simulink model "FOC_physical"  (R2024b)
settings: Solver=FixedStepAuto  StartTime=0.0  StopTime=3  FixedStep=1e-6  RelTol=1e-3
undefined symbols (not defined in the file): Down, GPTRIP1SEL, Ki_d, Ki_q, Ki_s, Kp_d, Kp_q, Kp_s, lambda, Ld, ma, p, T_max, TZ1, Up, Vdc
libraries: spsIGBTDiodeLib x6, simulink x4, spsCurrentMeasurementLib x3, spsDCVoltageSourceLib x1, spsPermanentMagnetSynchronousMachineLib x1, c2802xlib x1, eeStairGenerator x1, sps_lib x1
settings Model: Creator=ahmed  LastModifiedBy=ahmed
settings SolverCC: ZeroCrossAlgorithm=Adaptive
settings DebuggingCC: IgnoredZcDiagnostic=none

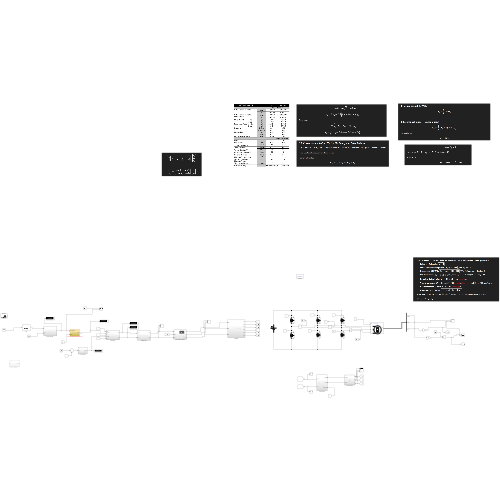
[thumbnail: Simulink's stored preview of the top-level diagram]
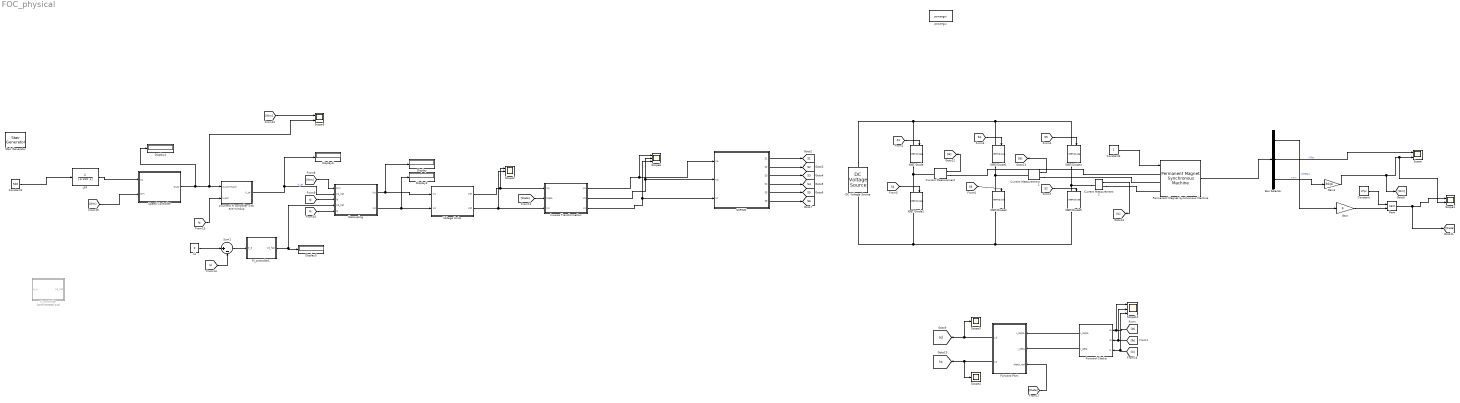
== system FOC_physical ==
  Bus Selector : BusSelector  OutputSignals=theta,Te,w
  Constant : Constant  Value=2*pi
  Constant1 : Constant  Value=500
  Constant3 : Constant
  Current Measurement : spsCurrentMeasurementLib/Current Measurement  PhasorSimulation=off  OutputType=Complex  PSBequivalent=0
  Current Measurement1 : spsCurrentMeasurementLib/Current Measurement  PhasorSimulation=off  OutputType=Complex  PSBequivalent=0
  Current Measurement2 : spsCurrentMeasurementLib/Current Measurement  PhasorSimulation=off  OutputType=Complex  PSBequivalent=0
  DC Voltage Source : spsDCVoltageSourceLib/DC Voltage Source  Amplitude=320  Measurements=None
  "Decoupling " : Subsystem
  Display{,3..6} (5 alike) : Display
  Forward Clacke : Subsystem
  Forward Park : Subsystem
  Gain : Gain  Gain=p
  Gain1 : Gain  Gain=30/pi
  IGBT/Diode{,1..5} (6 alike) : spsIGBTDiodeLib/IGBT//Diode  Ron=1e-3  Rs=1e5  Cs=inf  Measurements=on
  Id : Constant  Value=0
  Inverse Transformation : Subsystem
  LPF : TransferFcn  Denominator=[1/100 1]
  PI_controller : Subsystem  Commented=on
  PI_controller1 : Subsystem
  Permanent Magnet Synchronous Machine : spsPermanentMagnetSynchronousMachineLib/Permanent Magnet Synchronous Machine  NbPhases=3  FluxDistribution=Sinusoidal  RotorType=Round  MechanicalLoad=Torque Tm  PresetModel=No  ShowDetailedParameters=on  MeasurementBus=on  Resistance=1.45  Inductance=8.5e-3  dqInductances=[6.2e-3,6.2e-3]  La=6.2e-3  MachineConstant=Flux linkage established by magnets (V.s)  Flux=.0620  VoltageCst=44.9822  TorqueCst=0.372  Flat=120  Mechanical=[2.6e-5 9.55e-5 4 .03]  PolePairs=4  InitialConditions=[0,0, 0,0]  InitialConditions5ph=[0 0 0 0 0 0]  RefAngle=Aligned with phase A axis (original Park)  IterativeDiscreteModel=Trapezoidal non iterative  TsBlock=-1  TsPowergui=0
  Rem : Math  Operator=rem
  SVPWM : Subsystem
  Scope : Scope  NumInputPorts=2
  Scope1 : Scope  NumInputPorts=2
  Scope12 : Scope  NumInputPorts=3
  Scope2 : Scope  NumInputPorts=3
  Scope3 : Scope
  Scope4 : Scope
  Scope5 : Scope  NumInputPorts=2
  Scope6 : Scope  NumInputPorts=3
  "Speed Controller " : Subsystem
  Stair Generator : eeStairGenerator/Stair Generator  LabelModeActiveChoice=Discrete  TimeInput=[0 1 1.3 1.7 2 2.4]  AmplitudeInput=[200 1000 3000 4500 2000 0]  SampleTime=1e-6  RepeatPattern=off  OutDataTypeStr=double
      settings: LibrarySourceBlock=ee_sl_lib/General Control/Stair Generator
  Sum1 : Sum  Inputs=|+-
  Voltage limits : Subsystem
  powergui : sps_lib/powergui  Priority=1  SimulationMode=Continuous  SampleTime=1e-6  frequency=60  Iterations=50  frequencyindice=0  Pbase=100e6  ErrMax=1e-4  UnitsV=kV  UnitsW=MW  buscounter=0  FunctionMessages=off  echomessages=off  EnableUseOfTLC=off  CurrentSourceSwitches=off  DisableSnubberDevices=off  DisableRonSwitches=off  DisableVfSwitches=off  DisplayEquations=off  AutomaticDiscreteSolvers=off  SolverType=Tustin/Backward Euler (TBE)  Interpol=off  ExternalGateDelay=off  methode=off  Ts=100  x0status=blocks  SPID=on  SwTol=0  HookPort=off  NonlinearTolerance=1e-4  nMaxIteration=100  ContinueOnMaxIteration=off  RestoreLinks=warning  ResistiveCurrentMeasurement=off  Frange=[0:2:500]  Ylog=off  Xlog=on  ShowGrid=off  save=off  variable=ZData  structure=0  ZoomFFT=off  StartTime=0.0  cycles=1  DisplayStyle=1  fundamental=60  FreqAxis=off  MaxFrequency=1000  frequencyindicesteady=1  RmsSteady=1  display=off
  q-current PI controller with anti-windup : Subsystem
  tag scope: Id=global, Iq=global, S1=global, S2=global, S3=global, S4=global, S5=global, S6=global
  wires:
  Rem/1 -> Scope1/1, [theta]
  Permanent Magnet Synchronous Machine/1 -> Bus Selector/1
  Gain/1 -> Rem/2
  Constant/1 -> Rem/1
  [S3] -> IGBT/Diode1/1
  [S6] -> IGBT/Diode3/1
  [S5] -> IGBT/Diode4/1
  SVPWM/1(S1) -> [S1]
  SVPWM/2(S2) -> [S2]
  SVPWM/6(S6) -> [S6]
  SVPWM/4(S4) -> [S4]
  SVPWM/3(S3) -> [S3]
  SVPWM/5(S5) -> [S5]
  [S4] -> IGBT/Diode2/1
  [S1] -> IGBT/Diode/1
  [S2] -> IGBT/Diode5/1
  [Iq] -> "Decoupling "/5(Iq)
  "Decoupling "/2(Vd) -> Display3/1, Voltage limits/2(Vd)
  [Wm] -> Scope5/1
  Voltage limits/2(Vd*) -> Inverse Transformation/3(Vd), Scope2/2
  [Id] -> "Decoupling "/3(Id)
  PI_controller1/1(Vd_hat) -> "Decoupling "/4(Vd_hat), Display5/1
  Id/1 -> Sum1/1
  Inverse Transformation/1(Va) -> SVPWM/1(Va), Scope6/1
  Sum1/1 -> PI_controller1/1(e_d)
  "Decoupling "/1(Vq) -> Display/1, Voltage limits/1(Vq)
  Voltage limits/1(Vq*) -> Scope2/1, Inverse Transformation/1(Vq)
  "Speed Controller "/1(Out1) -> Display4/1, q-current PI controller with anti-windup/1(Iq command), Scope5/2
  Inverse Transformation/3(Vc) -> SVPWM/3(Vc), Scope6/3
  [theta] -> Inverse Transformation/2(theta)
  [Wm] -> "Decoupling "/1(Wm)
  Inverse Transformation/2(Vb) -> SVPWM/2(Vb), Scope6/2
  Constant3/1 -> Permanent Magnet Synchronous Machine/1
  [Id] -> Sum1/2
  [Wm] -> "Speed Controller "/2(Wm)
  Gain1/1 -> Scope1/2, Scope/2, [Wm]
  LPF/1 -> "Speed Controller "/1(In1)
  Forward Clacke/1(I_alpha) -> Forward Park/1(I_alpha)
  [theta] -> Forward Park/3(theta_rad)
  [Ib] -> Forward Clacke/2(Ib), Scope12/2
  Forward Park/1(I_d) -> [Id], Scope3/1
  [Ia] -> Forward Clacke/1(Ia), Scope12/1
  [Ic] -> Forward Clacke/3(Ic), Scope12/3
  Forward Park/2(I_q) -> [Iq], Scope4/1
  Forward Clacke/2(I_beta) -> Forward Park/2(I_beta)
  Current Measurement/1 -> [Ia]
  Current Measurement1/1 -> [Ib]
  Current Measurement2/1 -> [Ic]
  [Iq] -> q-current PI controller with anti-windup/2(Iq act)
  q-current PI controller with anti-windup/1(V_q*) -> Display6/1, "Decoupling "/2(Vq_hat)  "V_q*"
  Constant1/1 -> LPF/1
  Bus Selector/1 -> Gain/1  "<theta>"
  Bus Selector/2 -> Scope/1  "<Te>"
  Bus Selector/3 -> Gain1/1  "<w>"
  connections:
  DC Voltage Source/RConn1 -- IGBT/Diode4/LConn1 -- IGBT/Diode1/LConn1 -- IGBT/Diode/LConn1
  Current Measurement/LConn1 -- IGBT/Diode/RConn1 -- IGBT/Diode2/LConn1
  Current Measurement2/LConn1 -- IGBT/Diode4/RConn1 -- IGBT/Diode5/LConn1
  DC Voltage Source/LConn1 -- IGBT/Diode5/RConn1 -- IGBT/Diode3/RConn1 -- IGBT/Diode2/RConn1
  Current Measurement1/LConn1 -- IGBT/Diode1/RConn1 -- IGBT/Diode3/LConn1
  Current Measurement2/RConn1 -- Permanent Magnet Synchronous Machine/LConn3
  Current Measurement1/RConn1 -- Permanent Magnet Synchronous Machine/LConn2
  Current Measurement/RConn1 -- Permanent Magnet Synchronous Machine/LConn1

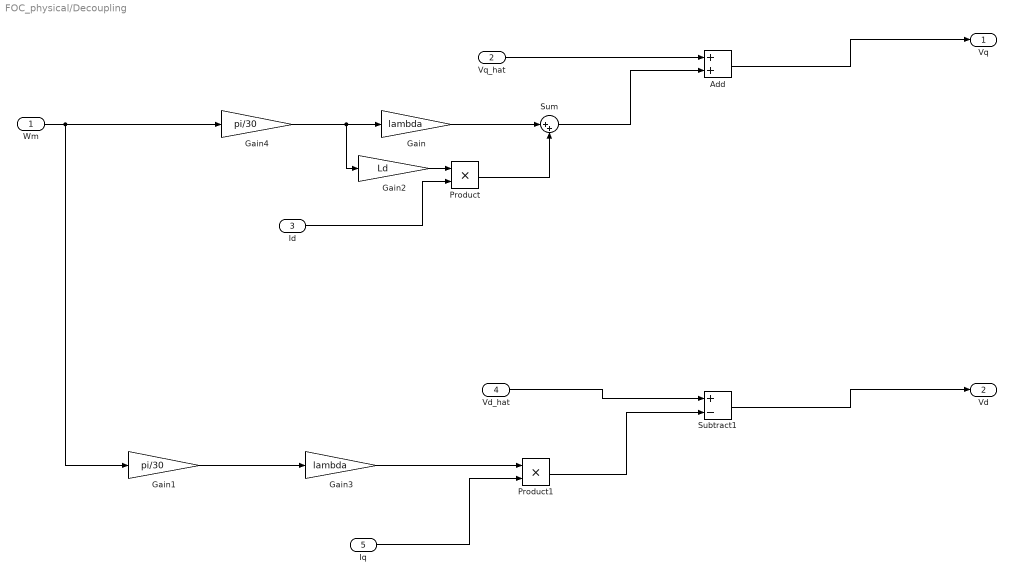
== system FOC_physical/Decoupling  ==
  Wm : Inport
  Vq_hat : Inport  Port=2
  Id : Inport  Port=3
  Vd_hat : Inport  Port=4
  Iq : Inport  Port=5
  Add : Sum
  Gain : Gain  Gain=lambda
  Gain1 : Gain  Gain=pi/30
  Gain2 : Gain  Gain=Ld
  Gain3 : Gain  Gain=lambda
  Gain4 : Gain  Gain=pi/30
  Product : Product
  Product1 : Product
  Subtract1 : Sum  Inputs=+-
  Sum : Sum  Inputs=|++
  Vq : Outport
  Vd : Outport  Port=2
  wires:
  Vq_hat/1 -> Add/1
  Vd_hat/1 -> Subtract1/1
  Gain2/1 -> Product/1
  Id/1 -> Product/2
  Product/1 -> Sum/2
  Gain/1 -> Sum/1
  Sum/1 -> Add/2
  Gain3/1 -> Product1/1
  Product1/1 -> Subtract1/2
  Iq/1 -> Product1/2
  Gain4/1 -> Gain2/1, Gain/1
  Add/1 -> Vq/1
  Subtract1/1 -> Vd/1
  Wm/1 -> Gain1/1, Gain4/1
  Gain1/1 -> Gain3/1

== system FOC_physical/Forward Clacke ==
  Ia : Inport
  Ib : Inport  Port=2
  Ic : Inport  Port=3
  Gain : Gain  Gain=0.5
  Gain1 : Gain  Gain=0.5
  Gain2 : Gain  Gain=2/3
  Gain3 : Gain  Gain=sqrt(3)/2
  Gain4 : Gain  Gain=2/3
  Sum : Sum  Inputs=+--
  Sum1 : Sum  Inputs=+-
  I_alpha : Outport
  I_beta : Outport  Port=2
  wires:
  Ib/1 -> Gain/1, Sum1/1
  Gain/1 -> Sum/2
  Gain2/1 -> I_alpha/1
  Sum1/1 -> Gain3/1
  Gain1/1 -> Sum/3
  Ic/1 -> Gain1/1, Sum1/2
  Sum/1 -> Gain2/1
  Gain3/1 -> Gain4/1
  Ia/1 -> Sum/1
  Gain4/1 -> I_beta/1

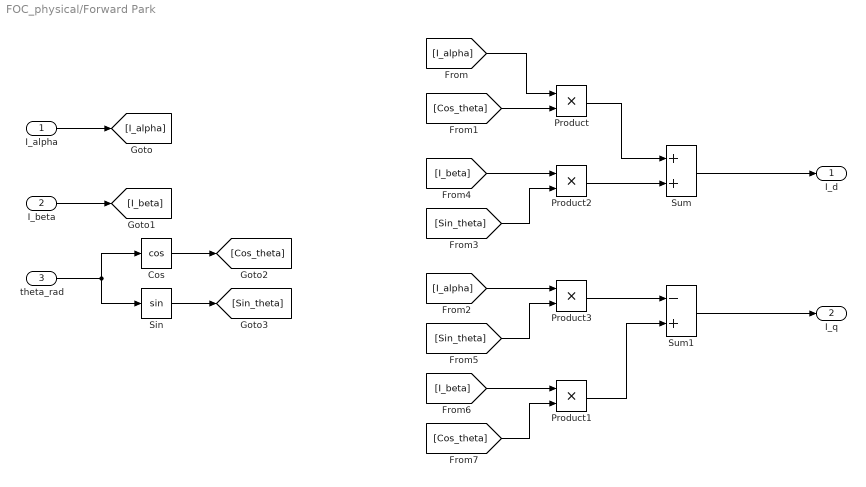
== system FOC_physical/Forward Park ==
  I_alpha : Inport
  I_beta : Inport  Port=2
  theta_rad : Inport  Port=3
  Cos : Trigonometry  Operator=cos
  Product{,1..3} (4 alike) : Product
  Sin : Trigonometry
  Sum : Sum
  Sum1 : Sum  Inputs=-+
  I_d : Outport
  I_q : Outport  Port=2
  wires:
  [Cos_theta] -> Product1/2
  [I_beta] -> Product1/1
  [Sin_theta] -> Product3/2
  [I_alpha] -> Product3/1
  Product1/1 -> Sum1/2
  [I_beta] -> Product2/1
  [Sin_theta] -> Product2/2
  [Cos_theta] -> Product/2
  Sin/1 -> [Sin_theta]
  Cos/1 -> [Cos_theta]
  theta_rad/1 -> Cos/1, Sin/1
  [I_alpha] -> Product/1
  I_beta/1 -> [I_beta]
  I_alpha/1 -> [I_alpha]
  Product3/1 -> Sum1/1
  Product2/1 -> Sum/2
  Product/1 -> Sum/1
  Sum1/1 -> I_q/1
  Sum/1 -> I_d/1

== system FOC_physical/Inverse Transformation ==
  Vq : Inport
  theta : Inport  Port=2
  Vd : Inport  Port=3
  "Inverse Park " : Subsystem
  inverse Clark : Subsystem
  Va : Outport
  Vb : Outport  Port=2
  Vc : Outport  Port=3
  wires:
  Vq/1 -> "Inverse Park "/3(In3)
  theta/1 -> "Inverse Park "/1(In1)
  Vd/1 -> "Inverse Park "/2(In2)
  "Inverse Park "/1(Valpha) -> inverse Clark/1(In1)
  "Inverse Park "/2(Vbeta) -> inverse Clark/2(In2)
  inverse Clark/1(Va) -> Va/1
  inverse Clark/2(Vb) -> Vb/1
  inverse Clark/3(Vc) -> Vc/1

== system FOC_physical/PI_controller ==
  note: Kp = ((2*zeta*wn)-(Rs/ld))*Ld
  note: Kp = (Wn^2)*Ld
  e_q : Inport
  Display : Display
  Integrator : Integrator
  Ki : Gain  Gain=Ki_q
  Kp : Gain  Gain=Kp_q
  Product : Product
  Scope : Scope
  Sum : Sum  Inputs=|++
  Vq_hat : Outport
  wires:
  Kp/1 -> Sum/1
  Sum/1 -> Display/1, Vq_hat/1
  e_q/1 -> Ki/1, Kp/1
  [Stop_q_integrator] -> Scope/1, Product/2
  Product/1 -> Integrator/1
  Integrator/1 -> Sum/2
  Ki/1 -> Product/1

== system FOC_physical/PI_controller1 ==
  e_d : Inport
  Integrator : Integrator
  Ki : Gain  Gain=Ki_d
  Kp : Gain  Gain=Kp_d
  Product : Product
  Sum : Sum  Inputs=|++
  Time Scope : Scope
  Vd_hat : Outport
  wires:
  Kp/1 -> Sum/1
  e_d/1 -> Ki/1, Kp/1
  Sum/1 -> Vd_hat/1
  Product/1 -> Integrator/1
  [Stop_d_integrator] -> Product/2, Time Scope/1
  Integrator/1 -> Sum/2
  Ki/1 -> Product/1

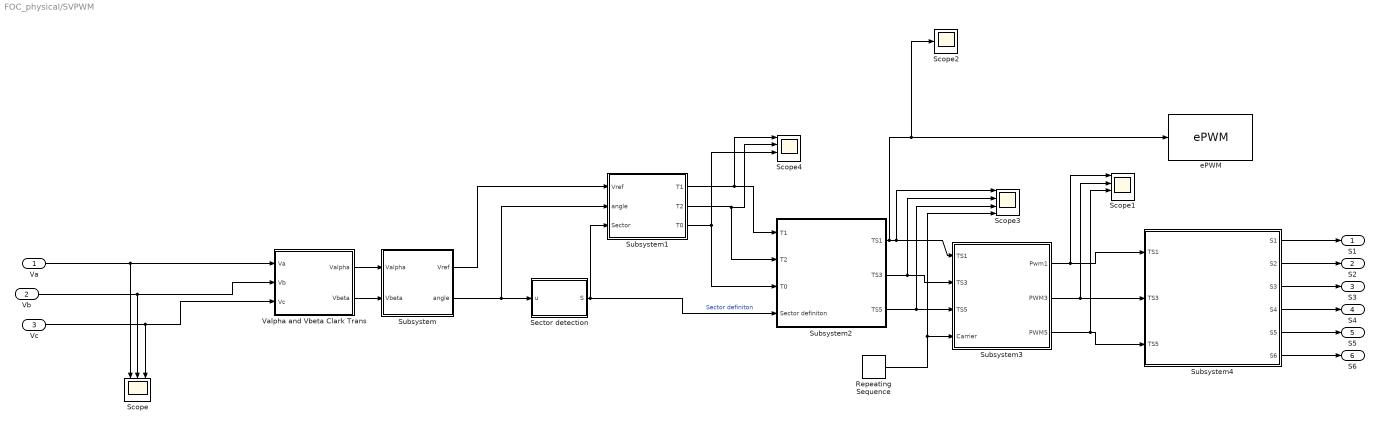
== system FOC_physical/SVPWM ==
  Va : Inport
  Vb : Inport  Port=2
  Vc : Inport  Port=3
  Repeating Sequence : simulink/Sources/Repeating Sequence  rep_seq_t=[0 1/20000 1/10000]  rep_seq_y=[0 1/1/10000 0]
  Scope : Scope  NumInputPorts=3
  Scope1 : Scope  NumInputPorts=4
  Scope2 : Scope
  Scope3 : Scope  NumInputPorts=4
  Scope4 : Scope  NumInputPorts=4
  Sector detection : MATLAB Function  TreatAsAtomicUnit=on
  Subsystem : Subsystem
  Subsystem1 : Subsystem
  Subsystem2 : Subsystem
  Subsystem3 : Subsystem
  Subsystem4 : Subsystem
  Valpha and Vbeta Clark Trans : Subsystem
  ePWM : c2802xlib/ePWM  PwmType=C2000_Type4  useModule=ePWM1  ePWMxLINKTBPRD=Not Linked  periodUnits=Clock cycles  timerSource=Specify via dialog  timerPeriod_clk=64000  timerPeriod_sec=0.0001  tbshadow=Counter equals to zero  countingMode=Up-Down  phaseActiveEnable=Disable  phaseDirection=Count down after sync  phaseActive=0  synchronizationEnable=off  dcaevt1Sync=off  dcbevt1Sync=off  synchronizationOption=Disable  dcbevt1SyncOut=off  dcaevt1SyncOut=off  cmpdSyncOut=off  cmpcSyncOut=off  cmpbSyncOut=off  zeroSyncOut=off  swfSyncOut=off  perSynchronizationOption=Counter equals to period (CTR=PRD)  clockPrescale=1  HSclockPrescale=1  enswap=off  ePWMxAStatus=on  ePWMxAactionLogic1=Do nothing  ePWMxAactionLogic2=Do nothing  ePWMxAactionLogic3=Clear  ePWMxAactionLogic4=Set  ePWMxAactionLogic5=Do nothing  ePWMxAactionLogic6=Do nothing  ePWMxACSFenable=off  ePWMxACSFvalue=Forcing disable  ePWMxASFreload=Zero  ePWMxBStatus=on  ePWMxBactionLogic1=Do nothing  ePWMxBactionLogic2=Do nothing  ePWMxBactionLogic3=Set  ePWMxBactionLogic4=Clear  ePWMxBactionLogic5=Do nothing  ePWMxBactionLogic6=Do nothing  ePWMxBCSFenable=off  ePWMxBCSFvalue=Forcing disable  ePWMxBSFreload=Zero  ePWNxBOutWay=off  ePWMxLINKCMPA=Not Linked  CMPAUnits=Percentages  CMPASource=Input port  CMPAValue_per=0  CMPAValue_clk=32000  enCMPAshadow=Counter equals to zero (CTR=Zero)  ePWMxLINKCMPB=Not Linked  CMPBUnits=Clock cycles  CMPBSource=Specify via dialog  CMPBValue_per=50  CMPBValue_clk=32000  enCMPBshadow=Counter equals to zero (CTR=Zero)  ePWMxLINKCMPC=Not Linked  CMPCUnits=Clock cycles  CMPCSource=Specify via dialog  CMPCValue_per=50  CMPCValue_clk=32000  enCMPCshadow=Counter equals to zero (CTR=Zero)  ePWMxLINKCMPD=Not Linked  CMPDUnits=Clock cycles  CMPDSource=Specify via dialog  CMPDValue_per=50  CMPDValue_clk=32000  enCMPDshadow=Counter equals to zero (CTR=Zero)  enableDBePWMxA=on  enableDBePWMxB=on  enhalfcycle=off  DBpolarity=Active high complementary (AHC)  DBedgeDelay=Positive  DBSource_ePWMxA=ePWMxA  DBSource_ePWMxB=ePWMxA  DBPeriodUnits=Seconds  DBperiodSource=Specify via dialog  REDperiod=0  FEDperiod=0  REDperiod_sec=1e-6  FEDperiod_sec=1e-6  LoadModeDBRED=Immediate without using shadow  LoadModeDBFED=Immediate without using shadow  adcstartModuleA=off  adcrequestEventA=First event  adcstartEventA=Digital Compare Module A Event 1 start of conversion (DCAEVT1.soc)  adcstartEventA_type2=Counter equals to zero (CTR=Zero)  adcstartModuleB=off  adcrequestEventB=First event  adcstartEventB=Counter equals to zero (CTR=Zero)  adcstartEventB_type2=Counter equals to zero (CTR=Zero)  intEn=off  intPrd=First event  intSel=Counter equals to zero (CTR=Zero)  intSel_type2=Counter equals to zero (CTR=Zero)  hrpe=off  enHRPWM=off  HRPWM_LoadMode=Counter equals to period (CTR=PRD)  HRPWM_CTLMode=Duty or Period control mode  HRPWM_EDGMode=Both edge  hrpeb=off  enHRPWMB=off  HRPWM_LoadModeB=Counter equals to zero (CTR=ZERO)  HRPWM_CTLModeB=Duty or Period control mode  HRPWM_EDGModeB=Both edge  enHRDBRED=off  enHRDBFED=off  enSFO=on  enautoconv=on  chopperEnable=off  chopperFrequency=1  chopperFirstwidth=1  chopperDuty=12.5%  tripZonesource=Specify via dialog  tzselOSHT1=off  tzselOSHT2=off  tzselOSHT3=off  tzselOSHT4=off  tzselOSHT5=off  tzselOSHT6=off  tzselOSHDCAEV1=off  tzselOSHDCBEV1=off  tzselCBC1=off  tzselCBC2=off  tzselCBC3=off  tzselCBC4=off  tzselCBC5=off  tzselCBC6=off  tzselCBCDCAEV2=off  tzselCBCDCBEV2=off  enTzOstIntr=off  enTzCbcIntr=off  enTzDCAEVT1Intr=off  enTzDCAEVT2Intr=off  enTzDCBEVT1Intr=off  enTzDCBEVT2Intr=off  tzclrCBCLatch=Counter equals to zero (CTR=Zero)  ePWMxAforced=No action  ePWMxBforced=No action  DCAEVT1forced=No action  DCBEVT1forced=No action  DCAEVT2forced=No action  DCBEVT2forced=No action  dcah=Trip Zone 1 input (TZ1)  dcal=Trip Zone 2 input (TZ2)  dcbh=Trip Zone 1 input (TZ1)  dcbl=Trip Zone 2 input (TZ2)  dcah_type2=GPTRIP1SEL/(TZ1)  dcal_type2=GPTRIP1SEL/(TZ1)  dcbh_type2=GPTRIP1SEL/(TZ1)  dcbl_type2=GPTRIP1SEL/(TZ1)  gendcaevt1=Event disabled  gendcaevt2=Event disabled  gendcbevt1=Event disabled  gendcbevt2=Event disabled  dcaevt1src=DCAEVT1 with sync  dcaevt2src=DCAEVT2 with sync  dcbevt1src=DCBEVT1 with sync  dcbevt2src=DCBEVT2 with sync  pulsesel=Counter equals to zero (CTR=Zero)  blankinv=off  blankoffset=0  blankwidth=0  evsrcsel=Filtered version of DCAEVT1 (DCAEVT1FILT)  encape=off
  S1 : Outport
  S2 : Outport  Port=2
  S3 : Outport  Port=3
  S4 : Outport  Port=4
  S5 : Outport  Port=5
  S6 : Outport  Port=6
  wires:
  Subsystem4/5(S5) -> S5/1
  Sector detection/1(S) -> Subsystem2/4(Sector definiton), Subsystem1/3(Sector)  "Sector definiton"
  Subsystem/2(angle) -> Sector detection/1(u), Subsystem1/2(angle)
  Subsystem/1(Vref) -> Subsystem1/1(Vref)
  Valpha and Vbeta Clark Trans/2(Vbeta) -> Subsystem/2(Vbeta)
  Va/1 -> Valpha and Vbeta Clark Trans/1(Va), Scope/1
  Repeating Sequence/1 -> Scope3/4, Subsystem3/4(Carrier)
  Valpha and Vbeta Clark Trans/1(Valpha) -> Subsystem/1(Valpha)
  Vb/1 -> Valpha and Vbeta Clark Trans/2(Vb), Scope/2
  Vc/1 -> Valpha and Vbeta Clark Trans/3(Vc), Scope/3
  Subsystem1/2(T2) -> Scope4/2, Subsystem2/2(T2)
  Subsystem1/1(T1) -> Scope4/1, Subsystem2/1(T1)
  Subsystem1/3(T0) -> Subsystem2/3(T0), Scope4/3
  Subsystem2/1(TS1) -> Scope2/1, ePWM/1, Subsystem3/1(TS1), Scope3/1
  Subsystem2/2(TS3) -> Subsystem3/2(TS3), Scope3/2
  Subsystem2/3(TS5) -> Subsystem3/3(TS5), Scope3/3
  Subsystem3/1(Pwm1) -> Scope1/1, Subsystem4/1(TS1)
  Subsystem3/2(PWM3) -> Scope1/2, Subsystem4/2(TS3)
  Subsystem3/3(PWM5) -> Scope1/3, Subsystem4/3(TS5)
  Subsystem4/1(S1) -> S1/1
  Subsystem4/2(S2) -> S2/1
  Subsystem4/3(S3) -> S3/1
  Subsystem4/4(S4) -> S4/1
  Subsystem4/6(S6) -> S6/1

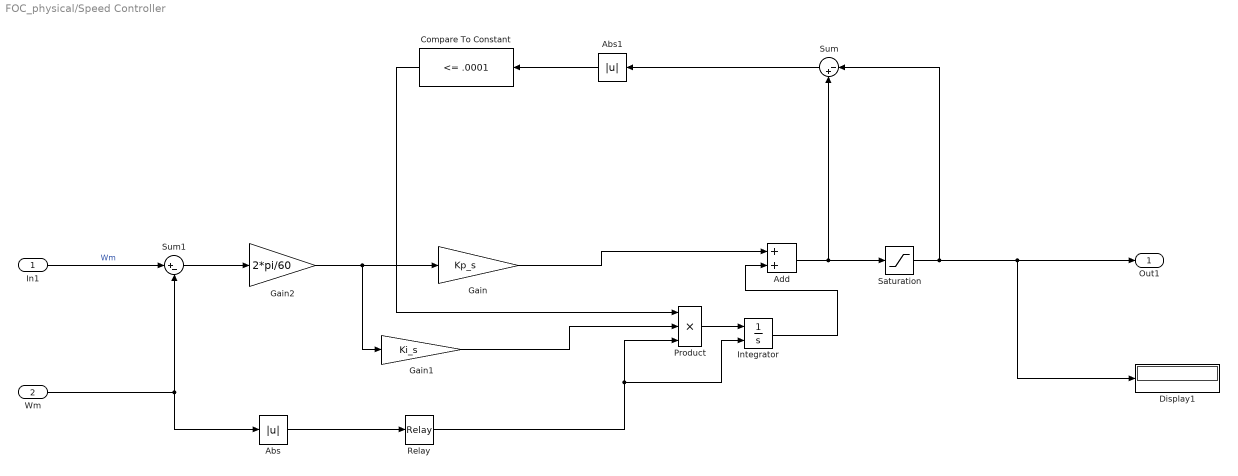
== system FOC_physical/Speed Controller  ==
  In1 : Inport
  Wm : Inport  Port=2
  Abs : Abs  SaturateOnIntegerOverflow=off
  Abs1 : Abs  SaturateOnIntegerOverflow=off
  Add : Sum
  Compare To Constant : simulink/Logic and Bit Operations/Compare To Constant  relop=<=  const=.0001  OutDataTypeStr=boolean
  Display1 : Display
  Gain : Gain  Gain=Kp_s
  Gain1 : Gain  Gain=Ki_s
  Gain2 : Gain  Gain=2*pi/60
  Integrator : Integrator  ExternalReset=falling
  Product : Product  Inputs=3
  Relay : Relay  OnSwitchValue=100  OffSwitchValue=-100
  Saturation : Saturate  UpperLimit=(2*T_max) / (3*p*lambda)  LowerLimit=0
  Sum : Sum  Inputs=|-+
  Sum1 : Sum  Inputs=|+-
  Out1 : Outport
  wires:
  Gain/1 -> Add/1
  Add/1 -> Saturation/1, Sum/2
  Gain2/1 -> Gain/1, Gain1/1
  In1/1 -> Sum1/1  "Wm"
  Wm/1 -> Abs/1, Sum1/2
  Sum1/1 -> Gain2/1
  Abs/1 -> Relay/1
  Product/1 -> Integrator/1
  Saturation/1 -> Sum/1, Out1/1, Display1/1
  Abs1/1 -> Compare To Constant/1
  Sum/1 -> Abs1/1
  Compare To Constant/1 -> Product/1
  Gain1/1 -> Product/2
  Relay/1 -> Integrator/2, Product/3
  Integrator/1 -> Add/2

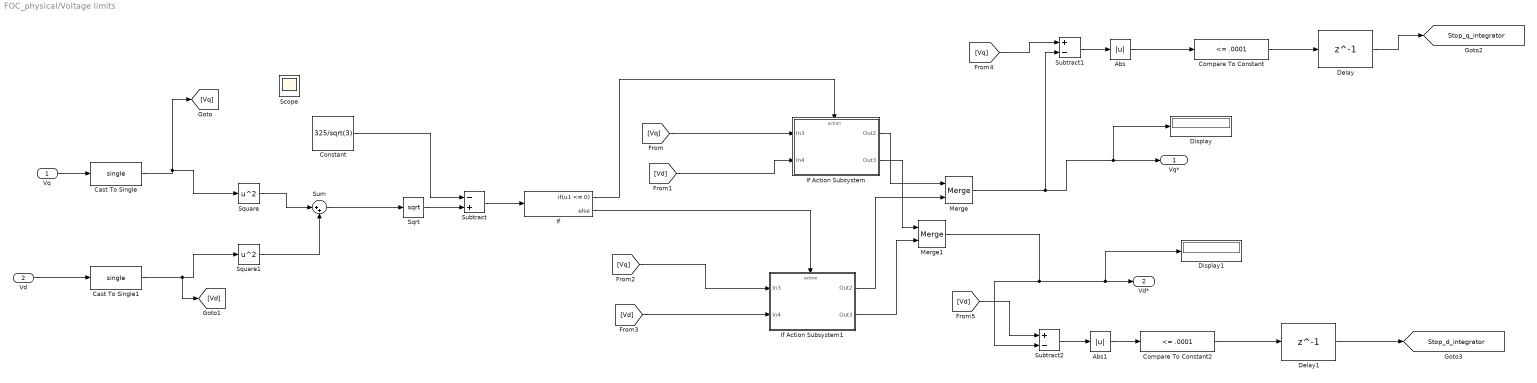
== system FOC_physical/Voltage limits ==
  Vq : Inport
  Vd : Inport  Port=2
  Abs : Abs  SaturateOnIntegerOverflow=off
  Abs1 : Abs  SaturateOnIntegerOverflow=off
  Cast To Single : DataTypeConversion  OutDataTypeStr=single  SaturateOnIntegerOverflow=off  RndMeth=Floor
  Cast To Single1 : DataTypeConversion  OutDataTypeStr=single  SaturateOnIntegerOverflow=off  RndMeth=Floor
  Compare To Constant : simulink/Logic and Bit Operations/Compare To Constant  relop=<=  const=.0001  OutDataTypeStr=boolean
  Compare To Constant2 : simulink/Logic and Bit Operations/Compare To Constant  relop=<=  const=.0001  OutDataTypeStr=boolean
  Constant : Constant  Value=325/sqrt(3)
  Delay : Delay  DelayLength=1
  Delay1 : Delay  DelayLength=1
  Display : Display
  Display1 : Display
  If : If  IfExpression=u1 <= 0
  If Action Subsystem : Subsystem  TreatAsAtomicUnit=on
  If Action Subsystem1 : Subsystem  TreatAsAtomicUnit=on
  Merge : Merge
  Merge1 : Merge
  Scope : Scope
  Sqrt : Sqrt
  Square : Math  Operator=square
  Square1 : Math  Operator=square
  Subtract : Sum  Inputs=-+
  Subtract1 : Sum  Inputs=+-
  Subtract2 : Sum  Inputs=+-
  Sum : Sum  Inputs=|++
  Vq* : Outport
  Vd* : Outport  Port=2
  tag scope: Stop_d_integrator=global, Stop_q_integrator=global
  wires:
  Vq/1 -> Cast To Single/1
  Vd/1 -> Cast To Single1/1
  Square/1 -> Sum/1
  Square1/1 -> Sum/2
  Sum/1 -> Sqrt/1
  Sqrt/1 -> Subtract/2
  Constant/1 -> Subtract/1
  Subtract/1 -> If/1
  If/1 -> If Action Subsystem/Action
  If/2 -> If Action Subsystem1/Action
  [Vq] -> If Action Subsystem/1(In3)
  [Vd] -> If Action Subsystem/2(In4)
  [Vq] -> If Action Subsystem1/1(In3)
  [Vd] -> If Action Subsystem1/2(In4)
  If Action Subsystem/1(Out2) -> Merge/1
  If Action Subsystem1/1(Out2) -> Merge/2
  If Action Subsystem/2(Out3) -> Merge1/1
  If Action Subsystem1/2(Out3) -> Merge1/2
  Merge/1 -> Subtract1/2, Display/1, Vq*/1
  Subtract1/1 -> Abs/1
  Abs/1 -> Compare To Constant/1
  Abs1/1 -> Compare To Constant2/1
  Subtract2/1 -> Abs1/1
  Compare To Constant/1 -> Delay/1
  Compare To Constant2/1 -> Delay1/1
  Delay/1 -> [Stop_q_integrator]
  Delay1/1 -> [Stop_d_integrator]
  Merge1/1 -> Subtract2/2, Display1/1, Vd*/1
  Cast To Single/1 -> [Vq], Square/1
  Cast To Single1/1 -> [Vd], Square1/1
  [Vq] -> Subtract1/1
  [Vd] -> Subtract2/1

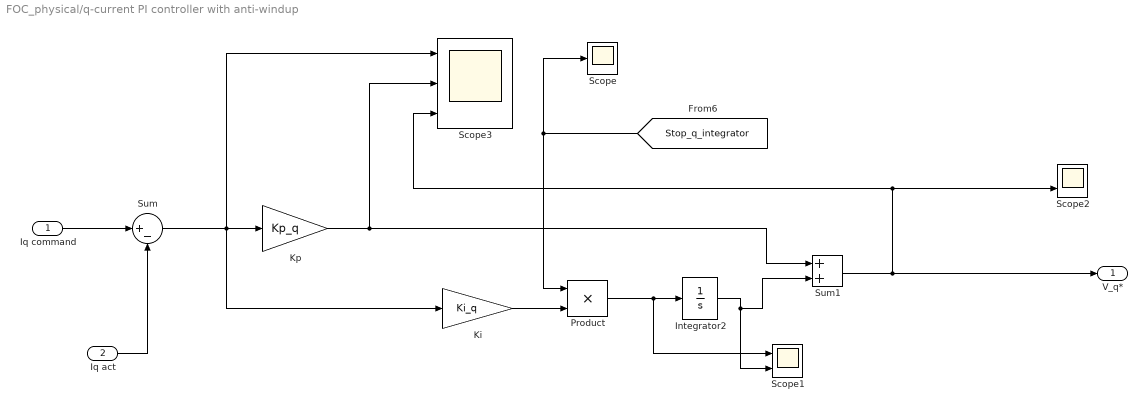
== system FOC_physical/q-current PI controller with anti-windup ==
  Iq command : Inport
  Iq act : Inport  Port=2
  Integrator2 : Integrator
  "Ki " : Gain  Gain=Ki_q
  Kp : Gain  Gain=Kp_q
  Product : Product
  Scope : Scope
  Scope1 : Scope  NumInputPorts=2
  Scope2 : Scope  NumInputPorts=2
  Scope3 : Scope  NumInputPorts=3
  Sum : Sum  Inputs=|+-
  Sum1 : Sum
  V_q* : Outport
  wires:
  Iq command/1 -> Sum/1
  Iq act/1 -> Sum/2
  Sum/1 -> "Ki "/1, Scope3/1, Kp/1
  Kp/1 -> Scope3/2, Sum1/1
  "Ki "/1 -> Product/2
  Product/1 -> Integrator2/1, Scope1/1
  Integrator2/1 -> Scope1/2, Sum1/2
  Sum1/1 -> V_q*/1, Scope2/2, Scope3/3
  [Stop_q_integrator] -> Scope/1, Product/1

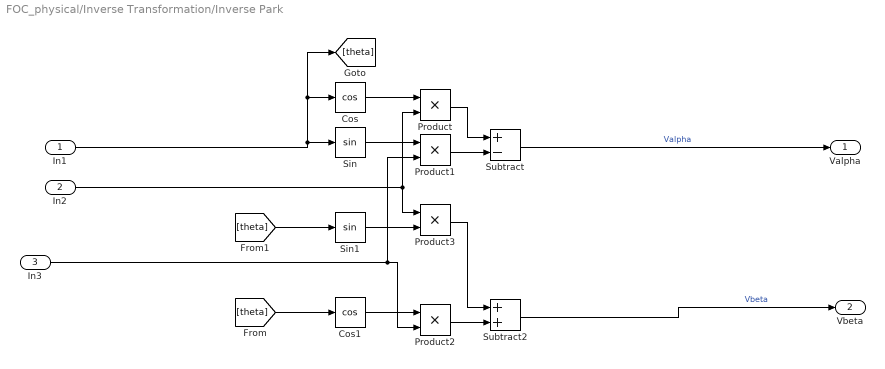
== system FOC_physical/Inverse Transformation/Inverse Park  ==
  In1 : Inport
  In2 : Inport  Port=2
  In3 : Inport  Port=3
  Cos : Trigonometry  Operator=cos
  Cos1 : Trigonometry  Operator=cos
  Product{,1..3} (4 alike) : Product
  Sin : Trigonometry
  Sin1 : Trigonometry
  Subtract : Sum  Inputs=+-
  Subtract2 : Sum
  Valpha : Outport
  Vbeta : Outport  Port=2
  wires:
  Product3/1 -> Subtract2/1
  In3/1 -> Product2/2, Product1/2
  In1/1 -> Cos/1, [theta], Sin/1
  Subtract/1 -> Valpha/1  "Valpha"
  Product/1 -> Subtract/1
  Subtract2/1 -> Vbeta/1  "Vbeta"
  Product2/1 -> Subtract2/2
  Cos/1 -> Product/1
  Product1/1 -> Subtract/2
  [theta] -> Cos1/1
  In2/1 -> Product/2, Product3/1
  [theta] -> Sin1/1
  Sin/1 -> Product1/1
  Cos1/1 -> Product2/1
  Sin1/1 -> Product3/2

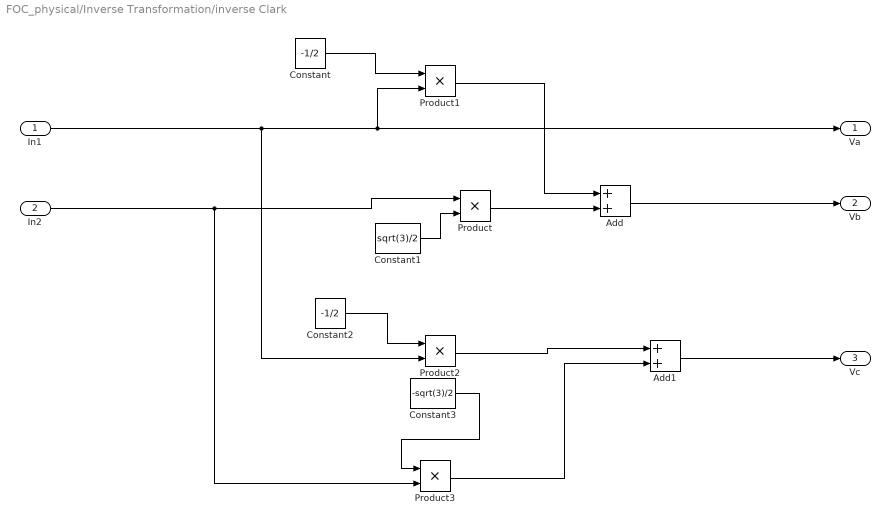
== system FOC_physical/Inverse Transformation/inverse Clark ==
  In1 : Inport
  In2 : Inport  Port=2
  Add : Sum
  Add1 : Sum
  Constant : Constant  Value=-1/2
  Constant1 : Constant  Value=sqrt(3)/2
  Constant2 : Constant  Value=-1/2
  Constant3 : Constant  Value=-sqrt(3)/2
  Product{,1..3} (4 alike) : Product
  Va : Outport
  Vb : Outport  Port=2
  Vc : Outport  Port=3
  wires:
  In1/1 -> Va/1, Product1/2, Product2/2
  In2/1 -> Product/1, Product3/2
  Add/1 -> Vb/1
  Product3/1 -> Add1/2
  Constant/1 -> Product1/1
  Constant2/1 -> Product2/1
  Product/1 -> Add/2
  Constant1/1 -> Product/2
  Product1/1 -> Add/1
  Product2/1 -> Add1/1
  Add1/1 -> Vc/1
  Constant3/1 -> Product3/1

== system FOC_physical/SVPWM/Subsystem ==
  Valpha : Inport
  Vbeta : Inport  Port=2
  Atan2 : Trigonometry  Operator=atan2
  Display : Display
  Display1 : Display
  Math Function : Math  Operator=square
  Math Function1 : Math  Operator=square
  Scope : Scope
  Sqrt1 : Sqrt
  Sum : Sum  Inputs=|++
  Vref : Outport
  angle : Outport  Port=2
  wires:
  Valpha/1 -> Atan2/2, Math Function/1
  Vbeta/1 -> Atan2/1, Math Function1/1
  Math Function/1 -> Sum/1
  Math Function1/1 -> Sum/2
  Sum/1 -> Sqrt1/1
  Sqrt1/1 -> Scope/1, Vref/1, Display/1
  Atan2/1 -> Display1/1, angle/1

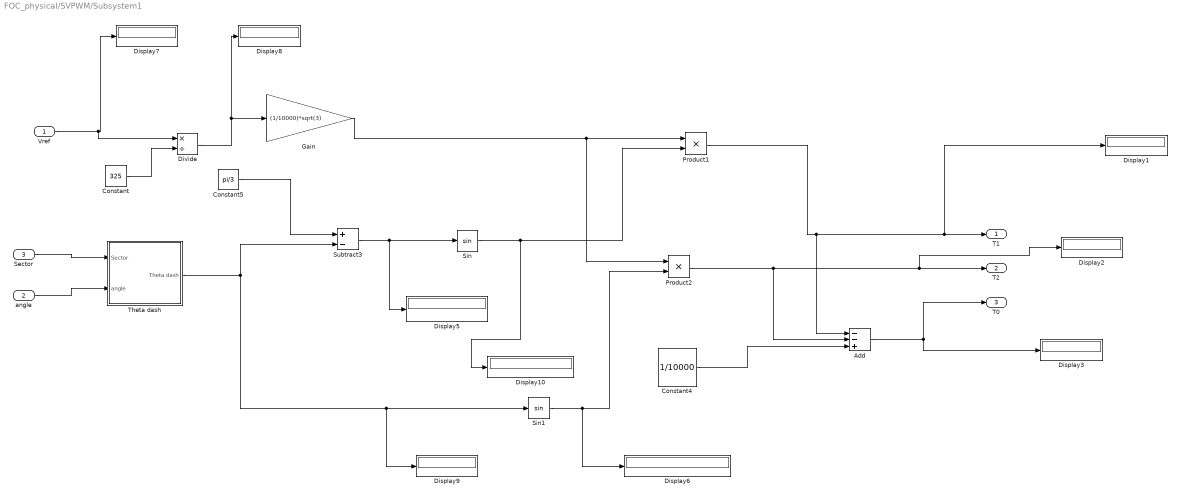
== system FOC_physical/SVPWM/Subsystem1 ==
  Vref : Inport
  angle : Inport  Port=2
  Sector : Inport  Port=3
  Add : Sum  Inputs=--+
  Constant : Constant  Value=325
  Constant4 : Constant  Value=1/10000
  Constant5 : Constant  Value=pi/3
  Display{1..3,5..10} (9 alike) : Display
  Divide : Product  Inputs=*/
  Gain : Gain  Gain=(1/10000)*sqrt(3)
  Product1 : Product
  Product2 : Product
  Sin : Trigonometry
  Sin1 : Trigonometry
  Subtract3 : Sum  Inputs=+-
  Theta dash : Subsystem
  T1 : Outport
  T2 : Outport  Port=2
  T0 : Outport  Port=3
  wires:
  Gain/1 -> Product2/1, Product1/1
  Product1/1 -> Display1/1, T1/1, Add/1
  Sin1/1 -> Display6/1, Product2/2
  Product2/1 -> Add/2, Display2/1, T2/1
  Constant4/1 -> Add/3
  Add/1 -> Display3/1, T0/1
  Constant5/1 -> Subtract3/1
  Subtract3/1 -> Sin/1, Display5/1
  Sin/1 -> Display10/1, Product1/2
  Divide/1 -> Display8/1, Gain/1
  Sector/1 -> Theta dash/1(Sector)
  angle/1 -> Theta dash/2(angle)
  Theta dash/1(Theta dash) -> Display9/1, Sin1/1, Subtract3/2
  Constant/1 -> Divide/2
  Vref/1 -> Divide/1, Display7/1

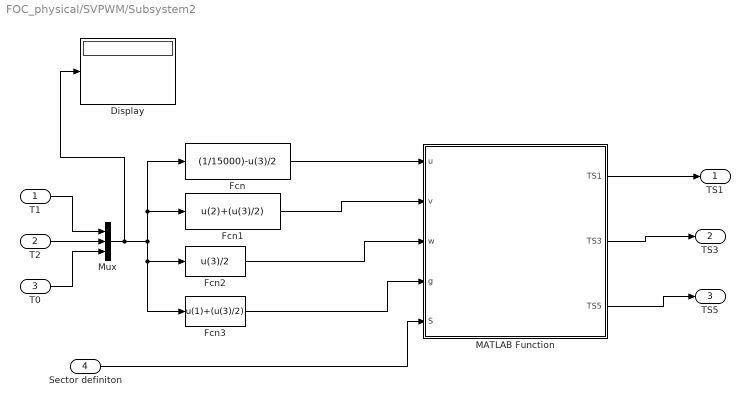
== system FOC_physical/SVPWM/Subsystem2 ==
  T1 : Inport
  T2 : Inport  Port=2
  T0 : Inport  Port=3
  Sector definiton : Inport  Port=4
  Display : Display
  Fcn : Fcn  Expr=(1/15000)-u(3)/2
  Fcn1 : Fcn  Expr=u(2)+(u(3)/2)
  Fcn2 : Fcn  Expr=u(3)/2
  Fcn3 : Fcn  Expr=u(1)+(u(3)/2)
  MATLAB Function : MATLAB Function  TreatAsAtomicUnit=on
  Mux : Mux  Inputs=3
  TS1 : Outport
  TS3 : Outport  Port=2
  TS5 : Outport  Port=3
  wires:
  MATLAB Function/1(TS1) -> TS1/1
  MATLAB Function/3(TS5) -> TS5/1
  MATLAB Function/2(TS3) -> TS3/1
  T1/1 -> Mux/1
  T2/1 -> Mux/2
  T0/1 -> Mux/3
  Mux/1 -> Display/1, Fcn1/1, Fcn/1, Fcn3/1, Fcn2/1
  Fcn/1 -> MATLAB Function/1(u)
  Fcn1/1 -> MATLAB Function/2(v)
  Fcn2/1 -> MATLAB Function/3(w)
  Fcn3/1 -> MATLAB Function/4(g)
  Sector definiton/1 -> MATLAB Function/5(S)

== system FOC_physical/SVPWM/Subsystem3 ==
  TS1 : Inport
  TS3 : Inport  Port=2
  TS5 : Inport  Port=3
  Carrier : Inport  Port=4
  Relational Operator : RelationalOperator  OutDataTypeStr=boolean  RndMeth=Simplest  InputSameDT=off
  Relational Operator1 : RelationalOperator  OutDataTypeStr=boolean  RndMeth=Simplest  InputSameDT=off
  Relational Operator2 : RelationalOperator  OutDataTypeStr=boolean  RndMeth=Simplest  InputSameDT=off
  Scope : Scope  NumInputPorts=3
  Pwm1 : Outport
  PWM3 : Outport  Port=2
  PWM5 : Outport  Port=3
  wires:
  TS1/1 -> Scope/1, Relational Operator/1
  TS3/1 -> Relational Operator1/1
  TS5/1 -> Relational Operator2/1
  Carrier/1 -> Scope/2, Relational Operator/2, Relational Operator1/2, Relational Operator2/2
  Relational Operator/1 -> Scope/3, Pwm1/1
  Relational Operator1/1 -> PWM3/1
  Relational Operator2/1 -> PWM5/1

== system FOC_physical/SVPWM/Subsystem4 ==
  TS1 : Inport
  TS3 : Inport  Port=2
  TS5 : Inport  Port=3
  NOT : Logic  Operator=NOT  IconShape=distinctive  AllPortsSameDT=off  OutDataTypeStr=boolean
  NOT1 : Logic  Operator=NOT  IconShape=distinctive  AllPortsSameDT=off  OutDataTypeStr=boolean
  NOT2 : Logic  Operator=NOT  IconShape=distinctive  AllPortsSameDT=off  OutDataTypeStr=boolean
  S1 : Outport
  S2 : Outport  Port=2
  S3 : Outport  Port=3
  S4 : Outport  Port=4
  S5 : Outport  Port=5
  S6 : Outport  Port=6
  wires:
  NOT2/1 -> S2/1
  TS5/1 -> NOT2/1, S5/1
  NOT1/1 -> S6/1
  TS3/1 -> S3/1, NOT1/1
  NOT/1 -> S4/1
  TS1/1 -> S1/1, NOT/1

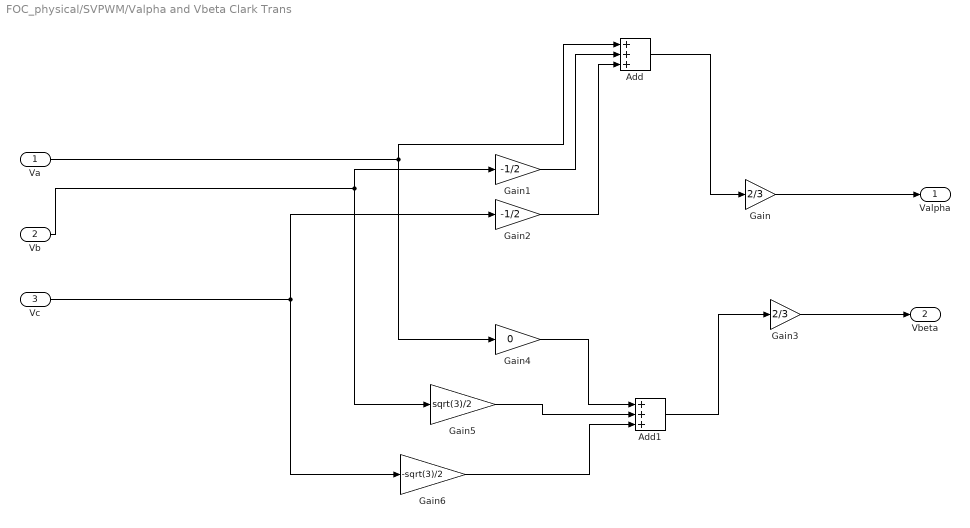
== system FOC_physical/SVPWM/Valpha and Vbeta Clark Trans ==
  Va : Inport
  Vb : Inport  Port=2
  Vc : Inport  Port=3
  Add : Sum  Inputs=+++
  Add1 : Sum  Inputs=+++
  Gain : Gain  Gain=2/3
  Gain1 : Gain  Gain=-1/2
  Gain2 : Gain  Gain=-1/2
  Gain3 : Gain  Gain=2/3
  Gain4 : Gain  Gain=0
  Gain5 : Gain  Gain=sqrt(3)/2
  Gain6 : Gain  Gain=-sqrt(3)/2
  Valpha : Outport
  Vbeta : Outport  Port=2
  wires:
  Va/1 -> Add/1, Gain4/1
  Vb/1 -> Gain5/1, Gain1/1
  Gain1/1 -> Add/2
  Vc/1 -> Gain2/1, Gain6/1
  Gain2/1 -> Add/3
  Add/1 -> Gain/1
  Gain4/1 -> Add1/1
  Gain5/1 -> Add1/2
  Gain6/1 -> Add1/3
  Add1/1 -> Gain3/1
  Gain/1 -> Valpha/1
  Gain3/1 -> Vbeta/1

== system FOC_physical/Voltage limits/If Action Subsystem ==
  In3 : Inport
  In4 : Inport  Port=2
  Action Port : ActionPort  ActionPortLabel=if(u1 <= 0)
  Out2 : Outport
  Out3 : Outport  Port=2
  wires:
  In3/1 -> Out2/1
  In4/1 -> Out3/1

== system FOC_physical/Voltage limits/If Action Subsystem1 ==
  In3 : Inport
  In4 : Inport  Port=2
  Action Port : ActionPort  ActionPortLabel=else
  Divide1 : Product  Inputs=*/  OutDataTypeStr=single
  Divide2 : Product  Inputs=/*  OutDataTypeStr=single
  Gain : Gain  Gain=sqrt(3)
  Gain1 : Gain  Gain=Vdc * ma
  Gain2 : Gain  Gain=Vdc * ma
  Square : Math  Operator=square  OutDataTypeStr=single
  Square Root : Sqrt  OutDataTypeStr=single  IntermediateResultsDataTypeStr=single
  Square1 : Math  Operator=square  OutDataTypeStr=single
  Sum : Sum  OutDataTypeStr=single  AccumDataTypeStr=single
  Out2 : Outport
  Out3 : Outport  Port=2
  wires:
  Divide1/1 -> Out2/1
  Divide2/1 -> Out3/1
  Square/1 -> Sum/1
  Sum/1 -> Square Root/1
  In3/1 -> Square/1, Gain1/1
  Gain2/1 -> Divide2/2
  Square1/1 -> Sum/2
  Square Root/1 -> Gain/1
  In4/1 -> Square1/1, Gain2/1
  Gain1/1 -> Divide1/1
  Gain/1 -> Divide2/1, Divide1/2

== system FOC_physical/SVPWM/Subsystem1/Theta dash ==
  Sector : Inport
  angle : Inport  Port=2
  Constant : Constant
  Display : Display
  Gain : Gain  Gain=(pi/3)
  Subtract : Sum  Inputs=-+
  Subtract1 : Sum  Inputs=-+
  Theta dash : Outport
  wires:
  angle/1 -> Subtract/2
  Gain/1 -> Subtract/1
  Constant/1 -> Subtract1/1
  Sector/1 -> Subtract1/2
  Subtract1/1 -> Gain/1
  Subtract/1 -> Display/1, Theta dash/1

== matlab function FOC_physical/SVPWM/Subsystem2/MATLAB Function ==
  data: TS1 output; u input; TS3 output; TS5 output; v input; w input; g input; S input
function [TS1, TS3,TS5] = fcn(u, v, w, g,S)

switch S
    case 1
        TS1 = u;
        TS3 = v;
        TS5 = w;
    case 2
        TS1 = g;
        TS3 = u;
        TS5 = w;
    case 3
        TS1 = w;
        TS3 = u;
        TS5 = v;
    case 4
        TS1 = w;
        TS3 = g;
        TS5 = u;
    case 5
        TS1 = v;
        TS3 = w;
        TS5 = u;
    case 6
        TS1 = u;
        TS3 = w;
        TS5 = g;
    otherwise
      TS1=0;  
      TS3=0;  
      TS5=0; 
end
end

== matlab function FOC_physical/SVPWM/Sector detection ==
  data: u input; S output
function S = fcn(u)

u = (180/pi)* u;

if(u < 60 && u >= 0)
    u = 1;
elseif(u < 120 && u >= 60)
    u = 2;
elseif(u < 180 && u >= 120)
    u = 3;
elseif(u < -120 && u >= -180)
u = 4;
elseif(u < -60 && u >= -120)
u = 5;
elseif(u < 0 && u >= -60)
u = 6;
else
    u = 0;
end
S = u;
